simulink model "mod_22"  (R2025a)
settings: Solver=ode45  StartTime=0.0  StopTime=10.0  MaxStep=1e-2  RelTol=1e-3
values from neighbouring files (symbols this model uses):
  a = 1000 + 1100*rand    [sistemas_lineales_iden.m]
  b = round(rand)    [sistemas_lineales_iden.m]
  c = 40 + 5*rand    [sistemas_lineales_iden.m]
  d = 100 + 50*rand    [sistemas_lineales_iden.m]
settings Model: Creator=fabri  LastModifiedBy=fabri

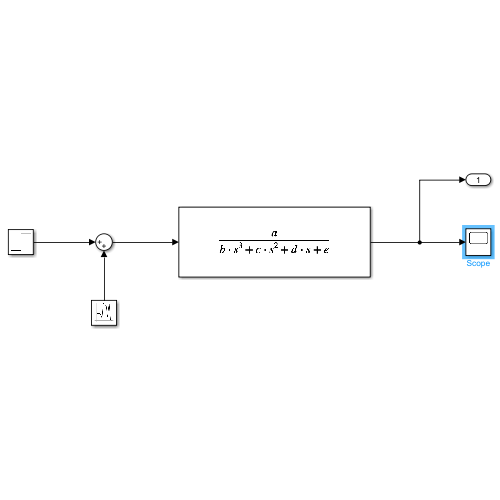
[thumbnail: Simulink's stored preview of the top-level diagram]
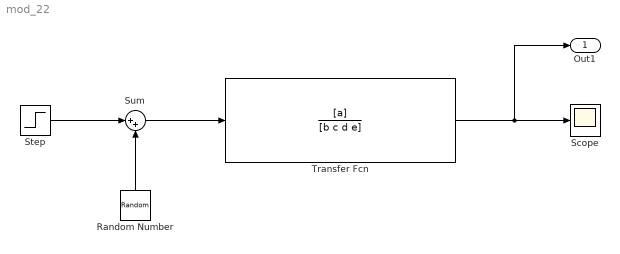
== system mod_22 ==
  Random Number : RandomNumber  Variance=0.01  SampleTime=0.1
  Scope : Scope
      settings: ActiveDisplayYMinimum=-0.17097424899152669  ActiveDisplayYMaximum=1.5387682409237404
  Step : Step  Time=0  SampleTime=0
  Sum : Sum  Inputs=|++
  Transfer Fcn : TransferFcn  Numerator=[a]  Denominator=[b c d e]
  Out1 : Outport
  wires:
  Transfer Fcn/1 -> Out1/1, Scope/1
  Random Number/1 -> Sum/2
  Step/1 -> Sum/1
  Sum/1 -> Transfer Fcn/1
